simulink model "ParId_Engine_Torque_and_Inertia"  (R2026b)
settings: Solver=VariableStepAuto
undefined symbols (not defined in the file): p_a, p_m, params
settings Model: Creator=User  LastModifiedBy=Mauro

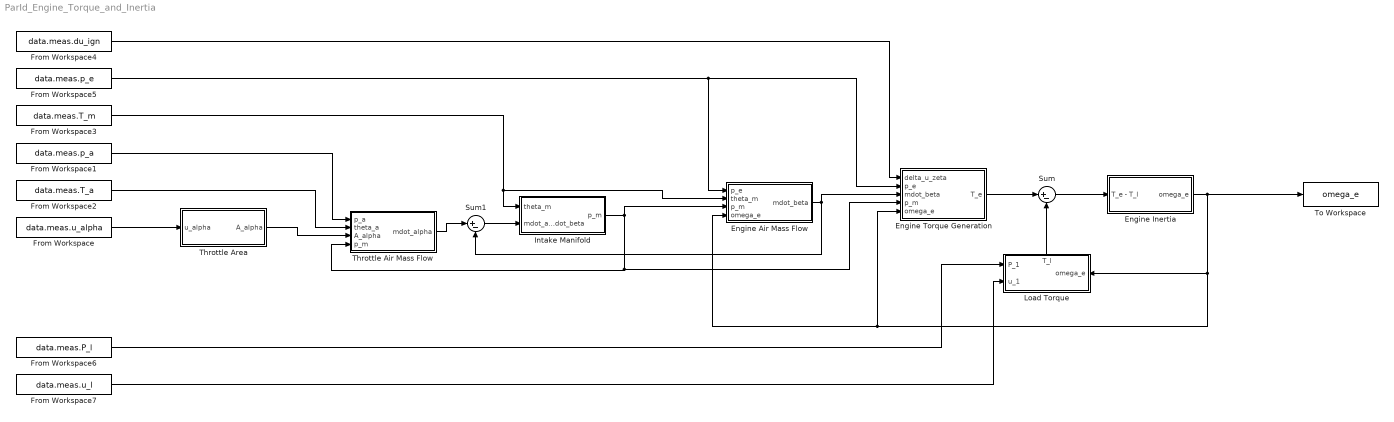
== system ParId_Engine_Torque_and_Inertia ==
  Engine Air Mass Flow : Subsystem
  Engine Inertia : Subsystem
  Engine Torque Generation : Subsystem
  From Workspace : FromWorkspace  VariableName=data.meas.u_alpha
  From Workspace1 : FromWorkspace  VariableName=data.meas.p_a
  From Workspace2 : FromWorkspace  VariableName=data.meas.T_a
  From Workspace3 : FromWorkspace  VariableName=data.meas.T_m
  From Workspace4 : FromWorkspace  VariableName=data.meas.du_ign
  From Workspace5 : FromWorkspace  VariableName=data.meas.p_e
  From Workspace6 : FromWorkspace  VariableName=data.meas.P_l
  From Workspace7 : FromWorkspace  VariableName=data.meas.u_l
  Intake Manifold : Subsystem
  Load Torque : Subsystem
      settings: PortSchema="{\"entries\":[{\"content\":{\"sides\":[{\"content\":{\"connectorIds\":[\"In1\",\"In2\"]},\"type\":\"ConnectorPlacement.EquallySpacedRectSide\",\"uuid\":\"2e69fc9b-1e0a-473f-9f43-16e3aff5faaf\"},{\"content\":{\"connectorIds\":[\"In3\"],\"side\":\"RIGHT\"},\"type\":\"ConnectorPlacement.EquallySpacedRectSide\",\"uuid\":\"22a941d9-30d8-4c58-89a5-97084a12a476\"},{\"content\":{\"connectorIds\":[\"Out1\"],\"side\":\"TOP\"},\"type\":\"ConnectorPlacement.EquallySpacedRectSide\",\"uuid\":\"512e319e-c2d4-4265-b8d2-2361f87cdc3a\"},{\"content\":{\"side\":\"BOTTOM\"},\"type\":\"ConnectorPlacement.EquallySpacedRectSide\",\"uuid\":\"2dcad07a-9bdb-41f9-89a6-3e027f1cf146\"}]},\"type\":\"ConnectorPlacement.EquallySpacedConnector\",\"uuid\":\"c866636f-332f-4d1f-a827-b340838fe4fa\"}],\"packageUris\":[\"http://schema.mathworks.com/mf0/Connector/R2020b\"],\"version\":\"1.0\"}"
  Sum : Sum  Inputs=|+-
  Sum1 : Sum  Inputs=|+-
  Throttle Air Mass Flow : Subsystem
  Throttle Area : Subsystem
  To Workspace : ToWorkspace  VariableName=omega_e  SaveFormat=Timeseries  SampleTime=-1
  wires:
  Engine Inertia/1(omega_e) -> To Workspace/1, Load Torque/3(omega_e), Engine Torque Generation/5(omega_e), Engine Air Mass Flow/4(omega_e)
  Throttle Area/1(A_alpha) -> Throttle Air Mass Flow/3(A_alpha)
  Sum1/1 -> Intake Manifold/2(mdot_alpha-mdot_beta)
  Sum/1 -> Engine Inertia/1(T_e - T_l)
  Load Torque/1(T_l) -> Sum/2
  Throttle Air Mass Flow/1(mdot_alpha) -> Sum1/1
  Intake Manifold/1(p_m) -> Engine Air Mass Flow/3(p_m), Engine Torque Generation/4(p_m), Throttle Air Mass Flow/4(p_m)
  Engine Air Mass Flow/1(mdot_beta) -> Engine Torque Generation/3(mdot_beta), Sum1/2
  Engine Torque Generation/1(T_e) -> Sum/1
  From Workspace2/1 -> Throttle Air Mass Flow/2(theta_a)
  From Workspace5/1 -> Engine Air Mass Flow/1(p_e), Engine Torque Generation/2(p_e)
  From Workspace3/1 -> Engine Air Mass Flow/2(theta_m), Intake Manifold/1(theta_m)
  From Workspace1/1 -> Throttle Air Mass Flow/1(p_a)
  From Workspace/1 -> Throttle Area/1(u_alpha)
  From Workspace4/1 -> Engine Torque Generation/1(delta_u_zeta)
  From Workspace6/1 -> Load Torque/1(P_1)
  From Workspace7/1 -> Load Torque/2(u_1)

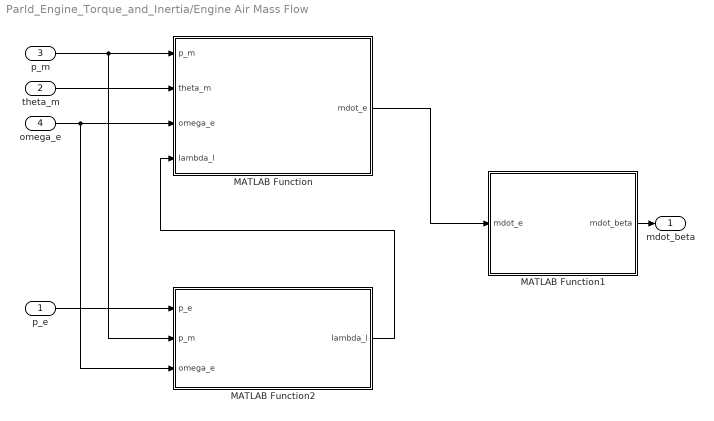
== system ParId_Engine_Torque_and_Inertia/Engine Air Mass Flow ==
  p_e : Inport
  theta_m : Inport  Port=2
  p_m : Inport  Port=3
  omega_e : Inport  Port=4
  MATLAB Function : MATLAB Function  TreatAsAtomicUnit=on
  MATLAB Function1 : MATLAB Function  TreatAsAtomicUnit=on
  MATLAB Function2 : MATLAB Function  TreatAsAtomicUnit=on
  mdot_beta : Outport
  wires:
  MATLAB Function2/1(lambda_l) -> MATLAB Function/4(lambda_l)
  MATLAB Function1/1(mdot_beta) -> mdot_beta/1
  theta_m/1 -> MATLAB Function/2(theta_m)
  p_e/1 -> MATLAB Function2/1(p_e)
  p_m/1 -> MATLAB Function2/2(p_m), MATLAB Function/1(p_m)
  MATLAB Function/1(mdot_e) -> MATLAB Function1/1(mdot_e)
  omega_e/1 -> MATLAB Function/3(omega_e), MATLAB Function2/3(omega_e)

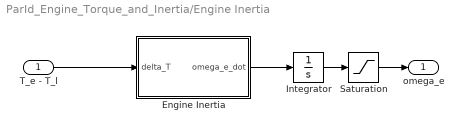
== system ParId_Engine_Torque_and_Inertia/Engine Inertia ==
  T_e - T_l : Inport
  Engine Inertia : MATLAB Function  TreatAsAtomicUnit=on
  Integrator : Integrator  InitialCondition=params.omega_e0
  Saturation : Saturate  UpperLimit=500  LowerLimit=20
  omega_e : Outport
  wires:
  T_e - T_l/1 -> Engine Inertia/1(delta_T)
  Engine Inertia/1(omega_e_dot) -> Integrator/1
  Integrator/1 -> Saturation/1
  Saturation/1 -> omega_e/1

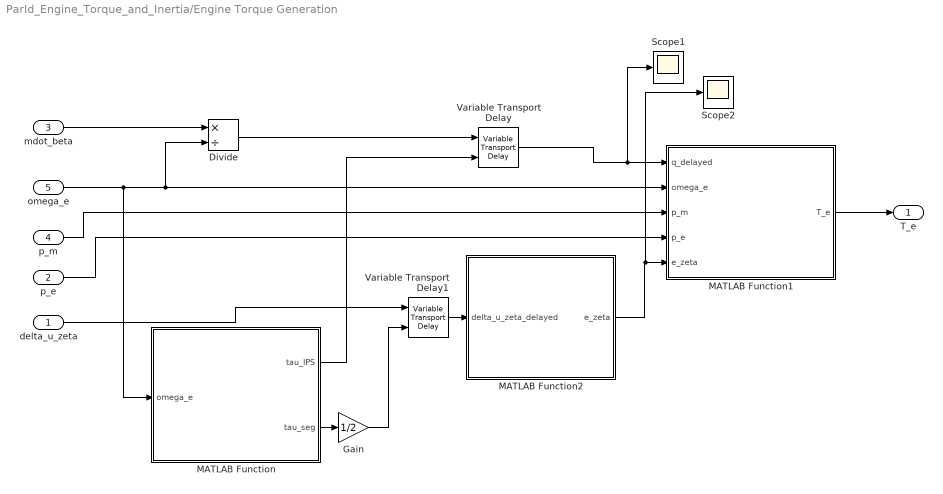
== system ParId_Engine_Torque_and_Inertia/Engine Torque Generation ==
  delta_u_zeta : Inport
  p_e : Inport  Port=2
  mdot_beta : Inport  Port=3
  p_m : Inport  Port=4
  omega_e : Inport  Port=5
  Divide : Product  Inputs=*/
  Gain : Gain  Gain=1/2
  MATLAB Function : MATLAB Function  TreatAsAtomicUnit=on
  MATLAB Function1 : MATLAB Function  TreatAsAtomicUnit=on
  MATLAB Function2 : MATLAB Function  TreatAsAtomicUnit=on
  Scope1 : Scope
      settings: ActiveDisplayYMinimum=-1  ActiveDisplayYMaximum=1
  Scope2 : Scope
      settings: ActiveDisplayYMinimum=-1  ActiveDisplayYMaximum=1  DataLoggingVariableName=ScopeData2
  Variable Transport Delay : VariableTransportDelay  MaximumDelay=10  MaximumPoints=16384
  Variable Transport Delay1 : VariableTransportDelay  MaximumDelay=10  MaximumPoints=16384
  T_e : Outport
  wires:
  p_m/1 -> MATLAB Function1/3(p_m)
  delta_u_zeta/1 -> Variable Transport Delay1/1
  omega_e/1 -> MATLAB Function1/2(omega_e), Divide/2, MATLAB Function/1(omega_e)
  Gain/1 -> Variable Transport Delay1/2
  MATLAB Function1/1(T_e) -> T_e/1
  mdot_beta/1 -> Divide/1
  Variable Transport Delay/1 -> Scope1/1, MATLAB Function1/1(q_delayed)
  MATLAB Function2/1(e_zeta) -> Scope2/1, MATLAB Function1/5(e_zeta)
  Divide/1 -> Variable Transport Delay/1
  p_e/1 -> MATLAB Function1/4(p_e)
  MATLAB Function/1(tau_IPS) -> Variable Transport Delay/2
  Variable Transport Delay1/1 -> MATLAB Function2/1(delta_u_zeta_delayed)
  MATLAB Function/2(tau_seg) -> Gain/1

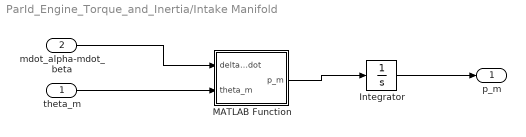
== system ParId_Engine_Torque_and_Inertia/Intake Manifold ==
  theta_m : Inport
  mdot_alpha-mdot_beta : Inport  Port=2
  Integrator : Integrator  InitialCondition=params.p_m0
  MATLAB Function : MATLAB Function  TreatAsAtomicUnit=on
  p_m : Outport
  wires:
  Integrator/1 -> p_m/1
  mdot_alpha-mdot_beta/1 -> MATLAB Function/1(delta_mdot)
  theta_m/1 -> MATLAB Function/2(theta_m)
  MATLAB Function/1(p_m) -> Integrator/1

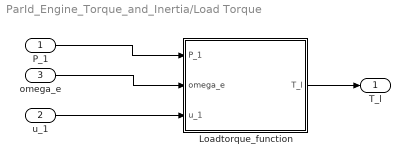
== system ParId_Engine_Torque_and_Inertia/Load Torque ==
  P_1 : Inport
  u_1 : Inport  Port=2
  omega_e : Inport  Port=3
  Loadtorque_function : MATLAB Function  TreatAsAtomicUnit=on
  T_l : Outport
  wires:
  u_1/1 -> Loadtorque_function/3(u_1)
  P_1/1 -> Loadtorque_function/1(P_1)
  Loadtorque_function/1(T_l) -> T_l/1
  omega_e/1 -> Loadtorque_function/2(omega_e)

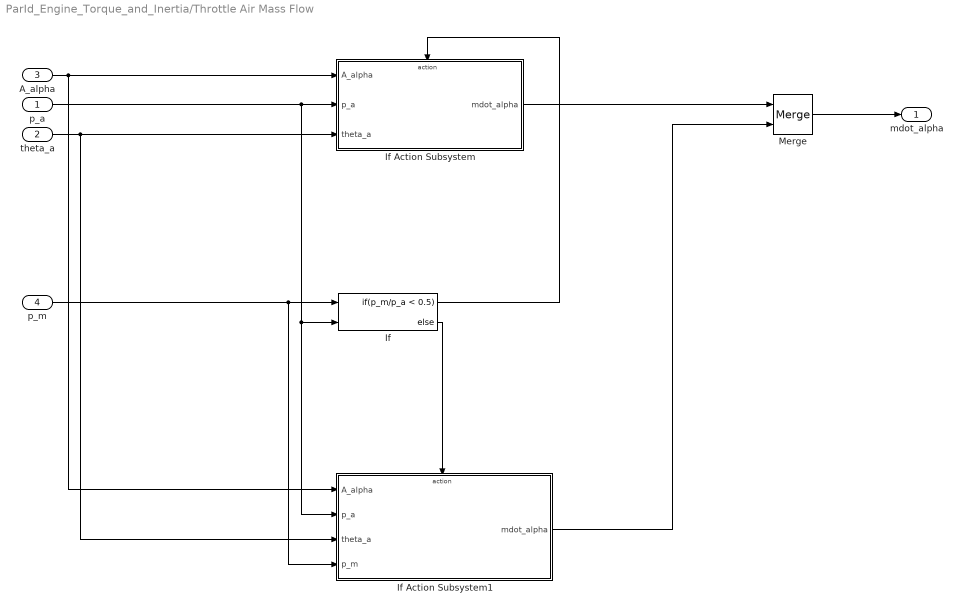
== system ParId_Engine_Torque_and_Inertia/Throttle Air Mass Flow ==
  p_a : Inport
  theta_a : Inport  Port=2
  A_alpha : Inport  Port=3
  p_m : Inport  Port=4
  If : If  NumInputs=2  IfExpression=p_m/p_a < 0.5  InportLabels=p_m,p_a
  If Action Subsystem : Subsystem  TreatAsAtomicUnit=on
  If Action Subsystem1 : Subsystem  TreatAsAtomicUnit=on
  Merge : Merge
  mdot_alpha : Outport
  wires:
  theta_a/1 -> If Action Subsystem/3(theta_a), If Action Subsystem1/3(theta_a)
  Merge/1 -> mdot_alpha/1
  If Action Subsystem/1(mdot_alpha) -> Merge/1
  p_a/1 -> If/2, If Action Subsystem1/2(p_a), If Action Subsystem/2(p_a)
  A_alpha/1 -> If Action Subsystem/1(A_alpha), If Action Subsystem1/1(A_alpha)
  If/2 -> If Action Subsystem1/Action
  If Action Subsystem1/1(mdot_alpha) -> Merge/2
  p_m/1 -> If/1, If Action Subsystem1/4(p_m)
  If/1 -> If Action Subsystem/Action

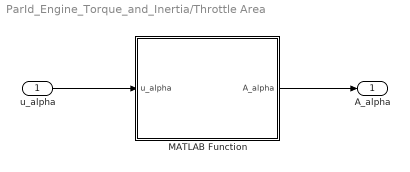
== system ParId_Engine_Torque_and_Inertia/Throttle Area ==
  u_alpha : Inport
  MATLAB Function : MATLAB Function  TreatAsAtomicUnit=on
  A_alpha : Outport
  wires:
  u_alpha/1 -> MATLAB Function/1(u_alpha)
  MATLAB Function/1(A_alpha) -> A_alpha/1

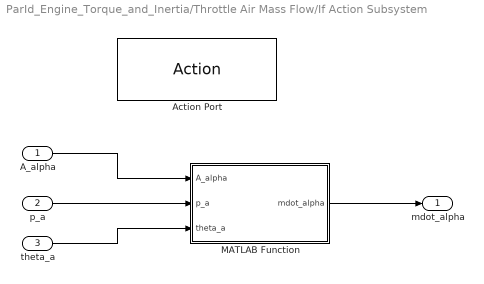
== system ParId_Engine_Torque_and_Inertia/Throttle Air Mass Flow/If Action Subsystem ==
  A_alpha : Inport
  p_a : Inport  Port=2
  theta_a : Inport  Port=3
  Action Port : ActionPort  ActionPortLabel=if(p_m/p_a < 0.5)
  MATLAB Function : MATLAB Function  TreatAsAtomicUnit=on
  mdot_alpha : Outport
  wires:
  A_alpha/1 -> MATLAB Function/1(A_alpha)
  p_a/1 -> MATLAB Function/2(p_a)
  theta_a/1 -> MATLAB Function/3(theta_a)
  MATLAB Function/1(mdot_alpha) -> mdot_alpha/1

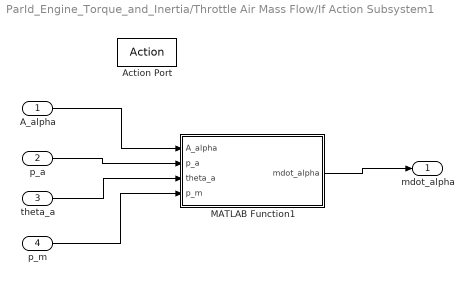
== system ParId_Engine_Torque_and_Inertia/Throttle Air Mass Flow/If Action Subsystem1 ==
  A_alpha : Inport
  p_a : Inport  Port=2
  theta_a : Inport  Port=3
  p_m : Inport  Port=4
  Action Port : ActionPort  ActionPortLabel=else
  MATLAB Function1 : MATLAB Function  TreatAsAtomicUnit=on
  mdot_alpha : Outport
  wires:
  A_alpha/1 -> MATLAB Function1/1(A_alpha)
  p_a/1 -> MATLAB Function1/2(p_a)
  theta_a/1 -> MATLAB Function1/3(theta_a)
  p_m/1 -> MATLAB Function1/4(p_m)
  MATLAB Function1/1(mdot_alpha) -> mdot_alpha/1

== matlab function ParId_Engine_Torque_and_Inertia/Engine Air Mass Flow/MATLAB Function ==
  data: mdot_e output; p_m input; theta_m input; omega_e input; lambda_l input; params parameter
function mdot_e = FreshMixtureMassFlow(p_m, theta_m, omega_e, lambda_l, params)

% Fresh mixture that enters the cylinder

mdot_e = 1/2 ... 
         * p_m/(params.R*theta_m) ...
         * lambda_l ...
         * params.V_d ... 
         * omega_e/(2*pi);

end

== matlab function ParId_Engine_Torque_and_Inertia/Engine Air Mass Flow/MATLAB Function1 ==
  data: mdot_beta output; mdot_e input; params parameter
function mdot_beta = MixtureToAirMassFlow(mdot_e, params)

% Air mass flow out of the intake manifold

mdot_beta = mdot_e / (1 + (1 / (params.lambda * params.sigma_0)));

end

== matlab function ParId_Engine_Torque_and_Inertia/Engine Air Mass Flow/MATLAB Function2 ==
  data: p_e input; lambda_l output; p_m input; omega_e input; params parameter
function lambda_l = VolumetricEfficiency(p_e, p_m, omega_e, params)

% Volumetric efficiency

lambda_lp = (params.V_c + params.V_d)/params.V_d ...
            - params.V_c/params.V_d ...
            * (p_e/p_m)^(1/params.kappa);

lambda_lomega = params.gamma_0 + params.gamma_1 * omega_e;

lambda_l = lambda_lp * lambda_lomega;

end

== matlab function ParId_Engine_Torque_and_Inertia/Load Torque/Loadtorque_function ==
  data: T_l output; P_1 input; omega_e input; u_1 input; params parameter
function T_l = fcn(P_1,omega_e,u_1, params)


T_l = u_1 * ...                             % probably multiply by u_1 since [1/0] on/off
      P_1 / (omega_e * params.eta_gen);

== matlab function ParId_Engine_Torque_and_Inertia/Intake Manifold/MATLAB Function ==
  data: delta_mdot input; theta_m input; p_m output; params parameter
function p_m = fcn(delta_mdot, theta_m, params)

p_m = delta_mdot * theta_m * params.R / params.Vm;

== matlab function ParId_Engine_Torque_and_Inertia/Throttle Air Mass Flow/If Action Subsystem/MATLAB Function ==
  data: A_alpha input; mdot_alpha output; p_a input; theta_a input; params parameter
function mdot_alpha = fcn(A_alpha,p_a,theta_a, params)

mdot_alpha = A_alpha * p_a/sqrt(params.R*theta_a) * 1/sqrt(2);

== matlab function ParId_Engine_Torque_and_Inertia/Throttle Air Mass Flow/If Action Subsystem1/MATLAB Function1 ==
  data: A_alpha input; mdot_alpha output; p_a input; theta_a input; p_m input; params parameter
function mdot_alpha = fcn(A_alpha, p_a, theta_a, p_m, params)

% if p_m/p_a >=1
%     mdot_alpha = 1;
%     fprintf('\nratio greater 1')
% else
%     mdot_alpha = A_alpha * p_a / sqrt(params.R * theta_a) * sqrt((2*p_m/p_a)*(1-p_m/p_a));
% end

mdot_alpha = A_alpha * p_a / sqrt(params.R * theta_a) * sqrt((2*p_m/p_a)*(1-p_m/p_a));

== matlab function ParId_Engine_Torque_and_Inertia/Engine Inertia/Engine Inertia ==
  data: delta_T input; omega_e_dot output; params parameter
function omega_e_dot = fcn(delta_T, params)

omega_e_dot = (1/params.theta_e)*(delta_T);

== matlab function ParId_Engine_Torque_and_Inertia/Engine Torque Generation/MATLAB Function ==
  data: omega_e input; tau_IPS output; tau_seg output
function [tau_IPS, tau_seg] = EngineDelayTimes(omega_e)

% the delays are defined as

tau_IPS = 2*pi / omega_e;      % time for one revolution

tau_seg = 4*pi / (5*omega_e);  % °CA intervals of combustion in one of the cylinders

end

== matlab function ParId_Engine_Torque_and_Inertia/Engine Torque Generation/MATLAB Function1 ==
  data: q_delayed input; omega_e input; p_m input; p_e input; e_zeta input; params parameter; T_e output
function T_e  = EngineTorque(q_delayed, omega_e, p_m, p_e, e_zeta, params)

% Torque produced by the engine

e_p_mphi = (params.eta_0 + params.eta_1*omega_e) ...
           * e_zeta * params.H_l/params.V_d ...
           * 4*pi/(params.lambda*params.sigma_0) ...
           * q_delayed;

p_me0f = params.beta_0 * 4*pi/params.V_d;

p_me0g = p_e - p_m;

p_me = e_p_mphi - p_me0f - p_me0g;

T_e = p_me * params.V_d/(4*pi);


end

== matlab function ParId_Engine_Torque_and_Inertia/Engine Torque Generation/MATLAB Function2 ==
  data: delta_u_zeta_delayed input; e_zeta output; params parameter
function e_zeta = IgnitionEfficiency(delta_u_zeta_delayed, params)

e_zeta = 1 - params.k_zeta * delta_u_zeta_delayed^2;

end

== matlab function ParId_Engine_Torque_and_Inertia/Throttle Area/MATLAB Function ==
  data: u_alpha input; A_alpha output; params parameter
function A_alpha = fcn(u_alpha, params)

A_alpha = params.alpha_0 + params.alpha_1*u_alpha;
